simulink model "gfm_pv_sil"  (R2018b)
settings: Solver=ode45  StartTime=0.0  StopTime=100  RelTol=1e-3
PreLoadFcn:
  | load_system('../simulink_reference_models/test_sequence_lib');
  | load_system('../simulink_reference_models/controls_element_lib');
InitFcn:
  | close all;
  | clear all;
  | clc;
  | 
  | % frequency nominals
  | F_NOM = 60;
  | W_NOM = 2 * pi * F_NOM;
  | 
  | C_DC = 40e-3;
  | V_LVDC_NOM = 1000;
  | 
  | % base values relative to inverter
  | % --------------------------------
  | VLL_INV_NOM = 480;
  | P_INV_NOM = 1e6;
  | Q_INV_NOM = 0.5e6;
  | S_INV_NOM = sqrt(P_INV_NOM^2 + Q_INV_NOM^2);
  | 
  | I_INV_BASE = S_INV_NOM/(sqrt(3)*VLL_INV_NOM);
  | Z_INV_BASE = VLL_INV_NOM^2/S_INV_NOM;
  | L_INV_BASE = Z_INV_BASE / W_NOM;
  | C_INV_BASE = 1 / (Z_INV_BASE * W_NOM);
  | 
  | % nominal ratings for power system model
  | % --------------------------------------
  | INVERTER_COUNT = 100;
  | 
  | VLV_NOM = VLL_INV_NOM;
  | VMV_NOM = 35e3;
  | VHV_NOM = 230e3;
  | S_PLANT = INVERTER_COUNT * S_INV_NOM;
  | 
  | N_GSU = VHV_NOM/VMV_NOM;
  | N_MVT = VMV_NOM/VLV_NOM;
  | 
  | I_LV_BASE = S_PLANT/(sqrt(3)*VLV_NOM);
  | I_MV_BASE = S_PLANT/(sqrt(3)*VMV_NOM);
  | I_HV_BASE = S_PLANT/(sqrt(3)*VHV_NOM);
  | 
  | Z_LV_BASE = VLV_NOM^2/S_PLANT;
  | Z_MV_BASE = VMV_NOM^2/S_PLANT;
  | Z_HV_BASE = VHV_NOM^2/S_PLANT;
  | 
  | L_LV_BASE = Z_LV_BASE / W_NOM;
  | L_MV_BASE = Z_MV_BASE / W_NOM;
  | L_HV_BASE = Z_HV_BASE / W_NOM;
  | C_LV_BASE = 1 / (Z_LV_BASE * W_NOM);
  | C_MV_BASE = 1 / (Z_MV_BASE * W_NOM);
  | C_HV_BASE = 1 / (Z_HV_BASE * W_NOM);
libraries: test_sequence_lib x14, controls_element_lib x2
settings Model: SimulationMode=accelerator  Creator=HussamAlatrash  LastModifiedBy=ahhei
settings DataIOCC: ReturnWorkspaceOutputs=on
settings DebuggingCC: UnconnectedInputMsg=none  UnconnectedOutputMsg=none  UnconnectedLineMsg=none
settings ModelReferenceCC: EnableRefExpFcnMdlSchedulingChecks=off
settings RTWCC: Description=Generic Real-Time Target
settings ConfigComp: CovBoundaryAbsTol=1.0e-5

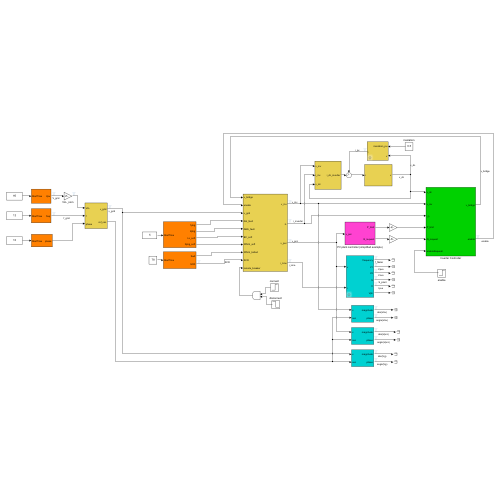
[thumbnail: Simulink's stored preview of the top-level diagram]
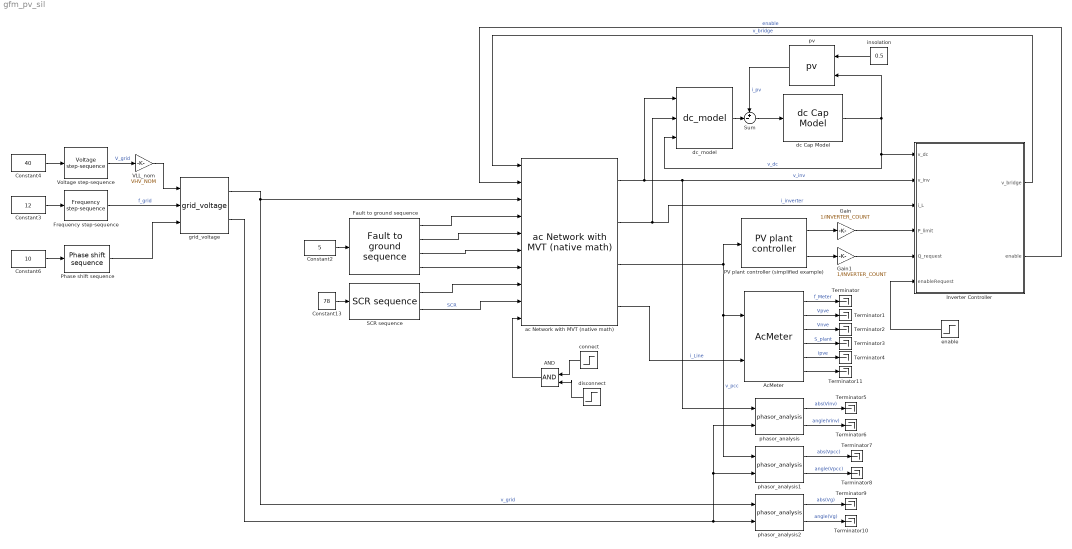
== system gfm_pv_sil ==
  AND : Logic  IconShape=distinctive  AllPortsSameDT=off  OutDataTypeStr=boolean
  AcMeter : test_sequence_lib/AcMeter  VllRated=VHV_NOM
  Constant13 : Constant  Value=78
  Constant2 : Constant  Value=5
  Constant3 : Constant  Value=12
  Constant4 : Constant  Value=40
  Constant6 : Constant  Value=10
  Fault to ground sequence : test_sequence_lib/Fault to ground sequence  SystemSampleTime=-1  EmptyChoice=off  PassThrough=off  PassThroughVariantControl=(default)  EmptyChoiceVariantControl=(default)  Latency=0  AutoFrameSizeCalculation=off
  Frequency step-sequence : test_sequence_lib/Frequency step-sequence  SystemSampleTime=-1  EmptyChoice=off  PassThrough=off  PassThroughVariantControl=(default)  EmptyChoiceVariantControl=(default)  Latency=0  AutoFrameSizeCalculation=off
  Gain : Gain  Gain=1/INVERTER_COUNT
  Gain1 : Gain  Gain=1/INVERTER_COUNT
  Inverter Controller : Subsystem
  PV plant controller (simplified example) : controls_element_lib/PV plant controller  SystemSampleTime=-1  EmptyChoice=off  PassThrough=off  PassThroughVariantControl=(default)  EmptyChoiceVariantControl=(default)  Latency=0  AutoFrameSizeCalculation=off
  Phase shift sequence : test_sequence_lib/Phase shift sequence  SystemSampleTime=-1  EmptyChoice=off  PassThrough=off  PassThroughVariantControl=(default)  EmptyChoiceVariantControl=(default)  Latency=0  AutoFrameSizeCalculation=off
  SCR sequence : test_sequence_lib/SCR sequence  SystemSampleTime=-1  EmptyChoice=off  PassThrough=off  PassThroughVariantControl=(default)  EmptyChoiceVariantControl=(default)  Latency=0  AutoFrameSizeCalculation=off
  Sum : Sum  Inputs=+-|
  Terminator{,1..11} (12 alike) : Terminator
  VLL_nom : Gain  Gain=VHV_NOM
  Voltage step-sequence : test_sequence_lib/Voltage step-sequence  SystemSampleTime=-1  EmptyChoice=off  PassThrough=off  PassThroughVariantControl=(default)  EmptyChoiceVariantControl=(default)  Latency=0  AutoFrameSizeCalculation=off
  ac Network with MVT (native math) : test_sequence_lib/ac Network with MVT (native math)  SystemSampleTime=-1  EmptyChoice=off  PassThrough=off  PassThroughVariantControl=(default)  EmptyChoiceVariantControl=(default)  Latency=0  AutoFrameSizeCalculation=off
  connect : Step  Time=0  SampleTime=0
  dc Cap Model : test_sequence_lib/dc Cap Model  SystemSampleTime=-1  EmptyChoice=off  PassThrough=off  PassThroughVariantControl=(default)  EmptyChoiceVariantControl=(default)  Latency=0  AutoFrameSizeCalculation=off
  dc_model : test_sequence_lib/dc_model  SystemSampleTime=-1  EmptyChoice=off  PassThrough=off  PassThroughVariantControl=(default)  EmptyChoiceVariantControl=(default)  Latency=0  AutoFrameSizeCalculation=off
  disconnect : Step  Time=97  Before=1  After=0  SampleTime=0
  enable : Step  Time=0.5  SampleTime=0
  grid_voltage : test_sequence_lib/grid_voltage  SystemSampleTime=-1  EmptyChoice=off  PassThrough=off  PassThroughVariantControl=(default)  EmptyChoiceVariantControl=(default)  Latency=0  AutoFrameSizeCalculation=off
  insolation : Constant  Value=0.5
  phasor_analysis : test_sequence_lib/phasor_analysis  SystemSampleTime=-1  EmptyChoice=off  PassThrough=off  PassThroughVariantControl=(default)  EmptyChoiceVariantControl=(default)  Latency=0  AutoFrameSizeCalculation=off
  phasor_analysis1 : test_sequence_lib/phasor_analysis  SystemSampleTime=-1  EmptyChoice=off  PassThrough=off  PassThroughVariantControl=(default)  EmptyChoiceVariantControl=(default)  Latency=0  AutoFrameSizeCalculation=off
  phasor_analysis2 : test_sequence_lib/phasor_analysis  SystemSampleTime=-1  EmptyChoice=off  PassThrough=off  PassThroughVariantControl=(default)  EmptyChoiceVariantControl=(default)  Latency=0  AutoFrameSizeCalculation=off
  pv : test_sequence_lib/pv  VopenCircuit=1500  IshortCircuit=1000
  wires:
  enable/1 -> Inverter Controller/6(enableRequest)
  Voltage step-sequence/1 -> VLL_nom/1  "V_grid"
  Gain1/1 -> Inverter Controller/5(Q_request)
  phasor_analysis1/2 -> Terminator8/1  "angle(Vpcc)"
  SCR sequence/2 -> ac Network with MVT (native math)/9  "SCR"
  Fault to ground sequence/4 -> ac Network with MVT (native math)/7
  AcMeter/1 -> Terminator/1  "f_Meter"
  Constant13/1 -> SCR sequence/1
  Gain/1 -> Inverter Controller/4(P_limit)
  VLL_nom/1 -> grid_voltage/1
  AcMeter/3 -> Terminator2/1  "Vnve"
  disconnect/1 -> AND/2
  Constant6/1 -> Phase shift sequence/1
  ac Network with MVT (native math)/3 -> PV plant controller (simplified example)/1, phasor_analysis1/1, AcMeter/1  "v_pcc"
  AcMeter/4 -> Terminator3/1  "S_plant"
  grid_voltage/1 -> ac Network with MVT (native math)/3, phasor_analysis2/1  "v_grid"
  insolation/1 -> pv/1
  AND/1 -> ac Network with MVT (native math)/10
  Constant4/1 -> Voltage step-sequence/1
  Constant2/1 -> Fault to ground sequence/1
  PV plant controller (simplified example)/1 -> Gain/1
  phasor_analysis2/1 -> Terminator9/1  "abs(Vg)"
  PV plant controller (simplified example)/2 -> Gain1/1
  phasor_analysis1/1 -> Terminator7/1  "abs(Vpcc)"
  Phase shift sequence/1 -> grid_voltage/3
  Fault to ground sequence/3 -> ac Network with MVT (native math)/6
  AcMeter/2 -> Terminator1/1  "Vpve"
  connect/1 -> AND/1
  Inverter Controller/2(enable) -> ac Network with MVT (native math)/2  "enable"
  AcMeter/6 -> Terminator11/1
  Constant3/1 -> Frequency step-sequence/1
  phasor_analysis/1 -> Terminator5/1  "abs(Vinv)"
  AcMeter/5 -> Terminator4/1  "Ipve"
  phasor_analysis/2 -> Terminator6/1  "angle(Vinv)"
  phasor_analysis2/2 -> Terminator10/1  "angle(Vg)"
  SCR sequence/1 -> ac Network with MVT (native math)/8
  Inverter Controller/1(v_bridge) -> ac Network with MVT (native math)/1  "v_bridge"
  Fault to ground sequence/1 -> ac Network with MVT (native math)/4
  grid_voltage/2 -> phasor_analysis1/2, phasor_analysis/2, phasor_analysis2/2
  ac Network with MVT (native math)/4 -> AcMeter/2  "i_Line"
  Frequency step-sequence/1 -> grid_voltage/2  "f_grid"
  Fault to ground sequence/2 -> ac Network with MVT (native math)/5
  ac Network with MVT (native math)/1 -> dc_model/1, Inverter Controller/2(v_inv), phasor_analysis/1  "v_inv"
  ac Network with MVT (native math)/2 -> dc_model/2, Inverter Controller/3(i_L)  "i_inverter"
  Sum/1 -> dc Cap Model/1
  dc Cap Model/1 -> pv/2, dc_model/3, Inverter Controller/1(v_dc)  "v_dc"
  dc_model/1 -> Sum/2
  pv/1 -> Sum/1  "i_pv"

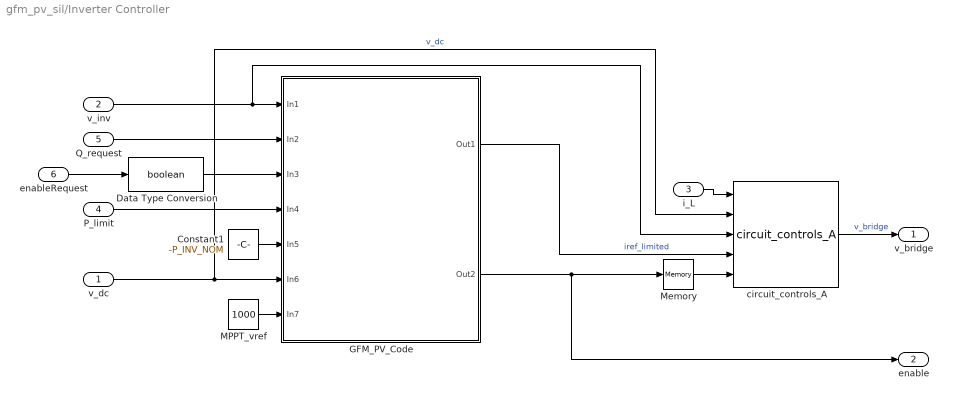
== system gfm_pv_sil/Inverter Controller ==
  v_dc : Inport
  v_inv : Inport  Port=2
  i_L : Inport  Port=3
  P_limit : Inport  Port=4
  Q_request : Inport  Port=5
  enableRequest : Inport  Port=6
  Constant1 : Constant  Value=-P_INV_NOM
  Data Type Conversion : DataTypeConversion  OutDataTypeStr=boolean
  GFM_PV_Code : Subsystem  Description=Replaced Block  mask(Replaced Block){}
      mask help: This block has been replaced with an empty subsystem because it used functionality that is unavailable in Simulink R2018b.
      mask Display: fprintf('Replaced: %s\n','CFunction')
  MPPT_vref : Constant  Value=1000
  Memory : Memory
  circuit_controls_A : controls_element_lib/circuit_controls_A  SystemSampleTime=-1  EmptyChoice=off  PassThrough=off  PassThroughVariantControl=(default)  EmptyChoiceVariantControl=(default)  Latency=0  AutoFrameSizeCalculation=off
  v_bridge : Outport
  enable : Outport  Port=2
  wires:
  circuit_controls_A/1 -> v_bridge/1  "v_bridge"
  v_inv/1 -> GFM_PV_Code/1(In1), circuit_controls_A/3
  GFM_PV_Code/1(Out1) -> circuit_controls_A/4  "iref_limited"
  v_dc/1 -> GFM_PV_Code/6(In6), circuit_controls_A/2  "v_dc"
  enableRequest/1 -> Data Type Conversion/1
  Q_request/1 -> GFM_PV_Code/2(In2)
  i_L/1 -> circuit_controls_A/1
  Constant1/1 -> GFM_PV_Code/5(In5)
  P_limit/1 -> GFM_PV_Code/4(In4)
  MPPT_vref/1 -> GFM_PV_Code/7(In7)
  Memory/1 -> circuit_controls_A/5
  Data Type Conversion/1 -> GFM_PV_Code/3(In3)
  GFM_PV_Code/2(Out2) -> Memory/1, enable/1

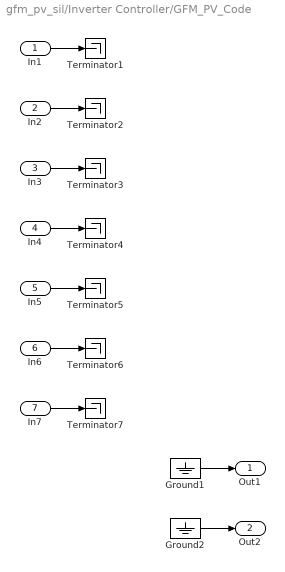
== system gfm_pv_sil/Inverter Controller/GFM_PV_Code ==
  In1 : Inport
  In2 : Inport  Port=2
  In3 : Inport  Port=3
  In4 : Inport  Port=4
  In5 : Inport  Port=5
  In6 : Inport  Port=6
  In7 : Inport  Port=7
  Ground1 : Ground
  Ground2 : Ground
  Terminator{1..7} (7 alike) : Terminator
  Out1 : Outport
  Out2 : Outport  Port=2
  wires:
  Ground2/1 -> Out2/1
  Ground1/1 -> Out1/1
  In7/1 -> Terminator7/1
  In6/1 -> Terminator6/1
  In5/1 -> Terminator5/1
  In4/1 -> Terminator4/1
  In3/1 -> Terminator3/1
  In2/1 -> Terminator2/1
  In1/1 -> Terminator1/1
